simulink model "My_gfm_battery_sil_1_BS_2"  (R2018b)
settings: Solver=ode23t  StartTime=0.0  StopTime=30  MaxStep=1e-4  RelTol=1e-3
PreLoadFcn:
  | modelDir = fileparts(get_param(bdroot,'FileName'));
  | 
  | load_system(fullfile(modelDir,'controls_element_lib.slx'));
  | load_system(fullfile(modelDir,'test_sequence_lib.slx'));
InitFcn:
  | close all;
  | clear all;
  | clc;
  | 
  | % frequency nominals
  | F_NOM = 60;
  | W_NOM = 2 * pi * F_NOM;
  | 
  | % base values relative to inverter
  | % --------------------------------
  | VLL_INV_NOM = 480;
  | P_INV_NOM = 1e6;
  | Q_INV_NOM = 0.5e6;
  | S_INV_NOM = sqrt(P_INV_NOM^2 + Q_INV_NOM^2);
  | 
  | I_INV_BASE = S_INV_NOM/(sqrt(3)*VLL_INV_NOM);
  | Z_INV_BASE = VLL_INV_NOM^2/S_INV_NOM;
  | L_INV_BASE = Z_INV_BASE / W_NOM;
  | C_INV_BASE = 1 / (Z_INV_BASE * W_NOM);
  | 
  | % nominal ratings for power system model
  | % --------------------------------------
  | INVERTER_COUNT = 100;
  | 
  | VLV_NOM = VLL_INV_NOM;
  | VMV_NOM = 35e3;
  | VHV_NOM = 230e3;
  | S_PLANT = INVERTER_COUNT * S_INV_NOM;
  | 
  | N_GSU = VHV_NOM/VMV_NOM;
  | N_MVT = VMV_NOM/VLV_NOM;
  | 
  | I_LV_BASE = S_PLANT/(sqrt(3)*VLV_NOM);
  | I_MV_BASE = S_PLANT/(sqrt(3)*VMV_NOM);
  | I_HV_BASE = S_PLANT/(sqrt(3)*VHV_NOM);
  | 
  | Z_LV_BASE = VLV_NOM^2/S_PLANT;
  | Z_MV_BASE = VMV_NOM^2/S_PLANT;
  | Z_HV_BASE = VHV_NOM^2/S_PLANT;
  | 
  | L_LV_BASE = Z_LV_BASE / W_NOM;
  | L_MV_BASE = Z_MV_BASE / W_NOM;
  | L_HV_BASE = Z_HV_BASE / W_NOM;
  | C_LV_BASE = 1 / (Z_LV_BASE * W_NOM);
  | C_MV_BASE = 1 / (Z_MV_BASE * W_NOM);
  | C_HV_BASE = 1 / (Z_HV_BASE * W_NOM);
undefined symbols (not defined in the file): j, kpFastSync, kpSync, kpSyncFade, SRated, SyncFadeThres, tauBkSt, VllRated, wSync
libraries: simulink x59, test_sequence_lib x9, controls_element_lib x8
(part 4 of 7)

== system My_gfm_battery_sil_1_BS_2/My Inverter Controller /My_acChecks_A_V1/OV3 Timer ==
  note: Min one sample delay on Rise
  note: Max one sample delay on Fall
  in : Inport
  Constant : Constant  Value=T_STEP
  Constant1 : Constant  Value=0
  Constant2 : Constant  Value=TIMEOUT
  Constant3 : Constant  Value=T_STEP
  Gain : Gain  Gain=0
  Min1 : MinMax  Function=max  Inputs=2
  Min2 : MinMax  Inputs=2
  Relational Operator : RelationalOperator  Operator=>  OutDataTypeStr=boolean  RndMeth=Simplest
  Sum1 : Sum  Inputs=|++
  Sum2 : Sum  Inputs=|++
  Switch : Switch  Criteria=u2 > Threshold
  Unit Delay : UnitDelay  SampleTime=T_STEP
  out : Outport  VectorParamsAs1DForOutWhenUnconnected=on
  wires:
  Sum2/1 -> Relational Operator/1, Min2/1
  Sum1/1 -> Min2/2, Relational Operator/2
  Constant/1 -> Sum2/1
  Min2/1 -> Switch/1
  Constant1/1 -> Switch/3
  Unit Delay/1 -> Sum2/2
  in/1 -> Switch/2
  Switch/1 -> Unit Delay/1
  Relational Operator/1 -> out/1
  Min1/1 -> Sum1/1
  Constant2/1 -> Min1/1
  Constant3/1 -> Min1/2, Gain/1
  Gain/1 -> Sum1/2

== system My_gfm_battery_sil_1_BS_2/My Inverter Controller /My_acChecks_A_V1/UF1 Timer ==
  note: Min one sample delay on Rise
  note: Max one sample delay on Fall
  in : Inport
  Constant : Constant  Value=T_STEP
  Constant1 : Constant  Value=0
  Constant2 : Constant  Value=TIMEOUT
  Constant3 : Constant  Value=T_STEP
  Gain : Gain  Gain=0
  Min1 : MinMax  Function=max  Inputs=2
  Min2 : MinMax  Inputs=2
  Relational Operator : RelationalOperator  Operator=>  OutDataTypeStr=boolean  RndMeth=Simplest
  Sum1 : Sum  Inputs=|++
  Sum2 : Sum  Inputs=|++
  Switch : Switch  Criteria=u2 > Threshold
  Unit Delay : UnitDelay  SampleTime=T_STEP
  out : Outport  VectorParamsAs1DForOutWhenUnconnected=on
  wires:
  Sum2/1 -> Relational Operator/1, Min2/1
  Sum1/1 -> Min2/2, Relational Operator/2
  Constant/1 -> Sum2/1
  Min2/1 -> Switch/1
  Constant1/1 -> Switch/3
  Unit Delay/1 -> Sum2/2
  in/1 -> Switch/2
  Switch/1 -> Unit Delay/1
  Relational Operator/1 -> out/1
  Min1/1 -> Sum1/1
  Constant2/1 -> Min1/1
  Constant3/1 -> Min1/2, Gain/1
  Gain/1 -> Sum1/2

== system My_gfm_battery_sil_1_BS_2/My Inverter Controller /My_acChecks_A_V1/UF2 Timer ==
  note: Min one sample delay on Rise
  note: Max one sample delay on Fall
  in : Inport
  Constant : Constant  Value=T_STEP
  Constant1 : Constant  Value=0
  Constant2 : Constant  Value=TIMEOUT
  Constant3 : Constant  Value=T_STEP
  Gain : Gain  Gain=0
  Min1 : MinMax  Function=max  Inputs=2
  Min2 : MinMax  Inputs=2
  Relational Operator : RelationalOperator  Operator=>  OutDataTypeStr=boolean  RndMeth=Simplest
  Sum1 : Sum  Inputs=|++
  Sum2 : Sum  Inputs=|++
  Switch : Switch  Criteria=u2 > Threshold
  Unit Delay : UnitDelay  SampleTime=T_STEP
  out : Outport  VectorParamsAs1DForOutWhenUnconnected=on
  wires:
  Sum2/1 -> Relational Operator/1, Min2/1
  Sum1/1 -> Min2/2, Relational Operator/2
  Constant/1 -> Sum2/1
  Min2/1 -> Switch/1
  Constant1/1 -> Switch/3
  Unit Delay/1 -> Sum2/2
  in/1 -> Switch/2
  Switch/1 -> Unit Delay/1
  Relational Operator/1 -> out/1
  Min1/1 -> Sum1/1
  Constant2/1 -> Min1/1
  Constant3/1 -> Min1/2, Gain/1
  Gain/1 -> Sum1/2

== system My_gfm_battery_sil_1_BS_2/My Inverter Controller /My_acChecks_A_V1/UF3 Timer ==
  note: Min one sample delay on Rise
  note: Max one sample delay on Fall
  in : Inport
  Constant : Constant  Value=T_STEP
  Constant1 : Constant  Value=0
  Constant2 : Constant  Value=TIMEOUT
  Constant3 : Constant  Value=T_STEP
  Gain : Gain  Gain=0
  Min1 : MinMax  Function=max  Inputs=2
  Min2 : MinMax  Inputs=2
  Relational Operator : RelationalOperator  Operator=>  OutDataTypeStr=boolean  RndMeth=Simplest
  Sum1 : Sum  Inputs=|++
  Sum2 : Sum  Inputs=|++
  Switch : Switch  Criteria=u2 > Threshold
  Unit Delay : UnitDelay  SampleTime=T_STEP
  out : Outport  VectorParamsAs1DForOutWhenUnconnected=on
  wires:
  Sum2/1 -> Relational Operator/1, Min2/1
  Sum1/1 -> Min2/2, Relational Operator/2
  Constant/1 -> Sum2/1
  Min2/1 -> Switch/1
  Constant1/1 -> Switch/3
  Unit Delay/1 -> Sum2/2
  in/1 -> Switch/2
  Switch/1 -> Unit Delay/1
  Relational Operator/1 -> out/1
  Min1/1 -> Sum1/1
  Constant2/1 -> Min1/1
  Constant3/1 -> Min1/2, Gain/1
  Gain/1 -> Sum1/2

== system My_gfm_battery_sil_1_BS_2/My Inverter Controller /My_acChecks_A_V1/UV1 Timer ==
  note: Min one sample delay on Rise
  note: Max one sample delay on Fall
  in : Inport
  Constant : Constant  Value=T_STEP
  Constant1 : Constant  Value=0
  Constant2 : Constant  Value=TIMEOUT
  Constant3 : Constant  Value=T_STEP
  Gain : Gain  Gain=0
  Min1 : MinMax  Function=max  Inputs=2
  Min2 : MinMax  Inputs=2
  Relational Operator : RelationalOperator  Operator=>  OutDataTypeStr=boolean  RndMeth=Simplest
  Sum1 : Sum  Inputs=|++
  Sum2 : Sum  Inputs=|++
  Switch : Switch  Criteria=u2 > Threshold
  Unit Delay : UnitDelay  SampleTime=T_STEP
  out : Outport  VectorParamsAs1DForOutWhenUnconnected=on
  wires:
  Sum2/1 -> Relational Operator/1, Min2/1
  Sum1/1 -> Min2/2, Relational Operator/2
  Constant/1 -> Sum2/1
  Min2/1 -> Switch/1
  Constant1/1 -> Switch/3
  Unit Delay/1 -> Sum2/2
  in/1 -> Switch/2
  Switch/1 -> Unit Delay/1
  Relational Operator/1 -> out/1
  Min1/1 -> Sum1/1
  Constant2/1 -> Min1/1
  Constant3/1 -> Min1/2, Gain/1
  Gain/1 -> Sum1/2

== system My_gfm_battery_sil_1_BS_2/My Inverter Controller /My_acChecks_A_V1/UV2 Timer ==
  note: Min one sample delay on Rise
  note: Max one sample delay on Fall
  in : Inport
  Constant : Constant  Value=T_STEP
  Constant1 : Constant  Value=0
  Constant2 : Constant  Value=TIMEOUT
  Constant3 : Constant  Value=T_STEP
  Gain : Gain  Gain=0
  Min1 : MinMax  Function=max  Inputs=2
  Min2 : MinMax  Inputs=2
  Relational Operator : RelationalOperator  Operator=>  OutDataTypeStr=boolean  RndMeth=Simplest
  Sum1 : Sum  Inputs=|++
  Sum2 : Sum  Inputs=|++
  Switch : Switch  Criteria=u2 > Threshold
  Unit Delay : UnitDelay  SampleTime=T_STEP
  out : Outport  VectorParamsAs1DForOutWhenUnconnected=on
  wires:
  Sum2/1 -> Relational Operator/1, Min2/1
  Sum1/1 -> Min2/2, Relational Operator/2
  Constant/1 -> Sum2/1
  Min2/1 -> Switch/1
  Constant1/1 -> Switch/3
  Unit Delay/1 -> Sum2/2
  in/1 -> Switch/2
  Switch/1 -> Unit Delay/1
  Relational Operator/1 -> out/1
  Min1/1 -> Sum1/1
  Constant2/1 -> Min1/1
  Constant3/1 -> Min1/2, Gain/1
  Gain/1 -> Sum1/2

== system My_gfm_battery_sil_1_BS_2/My Inverter Controller /My_acChecks_A_V1/UV3 Timer ==
  note: Min one sample delay on Rise
  note: Max one sample delay on Fall
  in : Inport
  Constant : Constant  Value=T_STEP
  Constant1 : Constant  Value=0
  Constant2 : Constant  Value=TIMEOUT
  Constant3 : Constant  Value=T_STEP
  Gain : Gain  Gain=0
  Min1 : MinMax  Function=max  Inputs=2
  Min2 : MinMax  Inputs=2
  Relational Operator : RelationalOperator  Operator=>  OutDataTypeStr=boolean  RndMeth=Simplest
  Sum1 : Sum  Inputs=|++
  Sum2 : Sum  Inputs=|++
  Switch : Switch  Criteria=u2 > Threshold
  Unit Delay : UnitDelay  SampleTime=T_STEP
  out : Outport  VectorParamsAs1DForOutWhenUnconnected=on
  wires:
  Sum2/1 -> Relational Operator/1, Min2/1
  Sum1/1 -> Min2/2, Relational Operator/2
  Constant/1 -> Sum2/1
  Min2/1 -> Switch/1
  Constant1/1 -> Switch/3
  Unit Delay/1 -> Sum2/2
  in/1 -> Switch/2
  Switch/1 -> Unit Delay/1
  Relational Operator/1 -> out/1
  Min1/1 -> Sum1/1
  Constant2/1 -> Min1/1
  Constant3/1 -> Min1/2, Gain/1
  Gain/1 -> Sum1/2

== system My_gfm_battery_sil_1_BS_2/My Inverter Controller /My_acChecks_A_V2/Assert Timer ==
  note: Min one sample delay on Rise
  note: Max one sample delay on Fall
  in : Inport
  Constant : Constant  Value=T_STEP
  Constant1 : Constant  Value=0
  Constant2 : Constant  Value=TIMEOUT
  Constant3 : Constant  Value=T_STEP
  Gain : Gain  Gain=0
  Min1 : MinMax  Function=max  Inputs=2
  Min2 : MinMax  Inputs=2
  Relational Operator : RelationalOperator  Operator=>  OutDataTypeStr=boolean  RndMeth=Simplest
  Sum1 : Sum  Inputs=|++
  Sum2 : Sum  Inputs=|++
  Switch : Switch  Criteria=u2 > Threshold
  Unit Delay : UnitDelay  SampleTime=T_STEP
  out : Outport  VectorParamsAs1DForOutWhenUnconnected=on
  wires:
  Sum2/1 -> Relational Operator/1, Min2/1
  Sum1/1 -> Min2/2, Relational Operator/2
  Constant/1 -> Sum2/1
  Min2/1 -> Switch/1
  Constant1/1 -> Switch/3
  Unit Delay/1 -> Sum2/2
  in/1 -> Switch/2
  Switch/1 -> Unit Delay/1
  Relational Operator/1 -> out/1
  Min1/1 -> Sum1/1
  Constant2/1 -> Min1/1
  Constant3/1 -> Min1/2, Gain/1
  Gain/1 -> Sum1/2

== system My_gfm_battery_sil_1_BS_2/My Inverter Controller /My_acChecks_A_V2/Clear Timer1 ==
  note: Max one sample delay on Rise
  note: Min one sample delay on Fall
  in : Inport
  Constant : Constant  Value=T_STEP
  Constant1 : Constant  Value=0
  Constant2 : Constant  Value=TIMEOUT
  Constant3 : Constant  Value=T_STEP
  Min1 : MinMax  Function=max  Inputs=2
  Min2 : MinMax  Function=max  Inputs=2
  Relational Operator : RelationalOperator  Operator=>  OutDataTypeStr=boolean  RndMeth=Simplest
  Sum1 : Sum  Inputs=|++
  Sum2 : Sum  Inputs=|-+
  Switch : Switch  Criteria=u2 > Threshold
  Unit Delay : UnitDelay  InitialCondition=TIMER_INIT  SampleTime=T_STEP
  out : Outport  VectorParamsAs1DForOutWhenUnconnected=on
  wires:
  Sum1/1 -> Switch/1
  Sum2/1 -> Relational Operator/1, Min2/1
  Constant/1 -> Sum2/1
  Min2/1 -> Switch/3
  Constant1/1 -> Min2/2, Relational Operator/2
  Unit Delay/1 -> Sum2/2
  in/1 -> Switch/2
  Switch/1 -> Unit Delay/1
  Relational Operator/1 -> out/1
  Constant2/1 -> Min1/1
  Constant3/1 -> Min1/2, Sum1/2
  Min1/1 -> Sum1/1

== system My_gfm_battery_sil_1_BS_2/My Inverter Controller /My_acChecks_A_V2/Clear Timer10 ==
  note: Max one sample delay on Rise
  note: Min one sample delay on Fall
  in : Inport
  Constant : Constant  Value=T_STEP
  Constant1 : Constant  Value=0
  Constant2 : Constant  Value=TIMEOUT
  Constant3 : Constant  Value=T_STEP
  Min1 : MinMax  Function=max  Inputs=2
  Min2 : MinMax  Function=max  Inputs=2
  Relational Operator : RelationalOperator  Operator=>  OutDataTypeStr=boolean  RndMeth=Simplest
  Sum1 : Sum  Inputs=|++
  Sum2 : Sum  Inputs=|-+
  Switch : Switch  Criteria=u2 > Threshold
  Unit Delay : UnitDelay  InitialCondition=TIMER_INIT  SampleTime=T_STEP
  out : Outport  VectorParamsAs1DForOutWhenUnconnected=on
  wires:
  Sum1/1 -> Switch/1
  Sum2/1 -> Relational Operator/1, Min2/1
  Constant/1 -> Sum2/1
  Min2/1 -> Switch/3
  Constant1/1 -> Min2/2, Relational Operator/2
  Unit Delay/1 -> Sum2/2
  in/1 -> Switch/2
  Switch/1 -> Unit Delay/1
  Relational Operator/1 -> out/1
  Constant2/1 -> Min1/1
  Constant3/1 -> Min1/2, Sum1/2
  Min1/1 -> Sum1/1

== system My_gfm_battery_sil_1_BS_2/My Inverter Controller /My_acChecks_A_V2/Clear Timer11 ==
  note: Max one sample delay on Rise
  note: Min one sample delay on Fall
  in : Inport
  Constant : Constant  Value=T_STEP
  Constant1 : Constant  Value=0
  Constant2 : Constant  Value=TIMEOUT
  Constant3 : Constant  Value=T_STEP
  Min1 : MinMax  Function=max  Inputs=2
  Min2 : MinMax  Function=max  Inputs=2
  Relational Operator : RelationalOperator  Operator=>  OutDataTypeStr=boolean  RndMeth=Simplest
  Sum1 : Sum  Inputs=|++
  Sum2 : Sum  Inputs=|-+
  Switch : Switch  Criteria=u2 > Threshold
  Unit Delay : UnitDelay  InitialCondition=TIMER_INIT  SampleTime=T_STEP
  out : Outport  VectorParamsAs1DForOutWhenUnconnected=on
  wires:
  Sum1/1 -> Switch/1
  Sum2/1 -> Relational Operator/1, Min2/1
  Constant/1 -> Sum2/1
  Min2/1 -> Switch/3
  Constant1/1 -> Min2/2, Relational Operator/2
  Unit Delay/1 -> Sum2/2
  in/1 -> Switch/2
  Switch/1 -> Unit Delay/1
  Relational Operator/1 -> out/1
  Constant2/1 -> Min1/1
  Constant3/1 -> Min1/2, Sum1/2
  Min1/1 -> Sum1/1

== system My_gfm_battery_sil_1_BS_2/My Inverter Controller /My_acChecks_A_V2/Clear Timer12 ==
  note: Max one sample delay on Rise
  note: Min one sample delay on Fall
  in : Inport
  Constant : Constant  Value=T_STEP
  Constant1 : Constant  Value=0
  Constant2 : Constant  Value=TIMEOUT
  Constant3 : Constant  Value=T_STEP
  Min1 : MinMax  Function=max  Inputs=2
  Min2 : MinMax  Function=max  Inputs=2
  Relational Operator : RelationalOperator  Operator=>  OutDataTypeStr=boolean  RndMeth=Simplest
  Sum1 : Sum  Inputs=|++
  Sum2 : Sum  Inputs=|-+
  Switch : Switch  Criteria=u2 > Threshold
  Unit Delay : UnitDelay  InitialCondition=TIMER_INIT  SampleTime=T_STEP
  out : Outport  VectorParamsAs1DForOutWhenUnconnected=on
  wires:
  Sum1/1 -> Switch/1
  Sum2/1 -> Relational Operator/1, Min2/1
  Constant/1 -> Sum2/1
  Min2/1 -> Switch/3
  Constant1/1 -> Min2/2, Relational Operator/2
  Unit Delay/1 -> Sum2/2
  in/1 -> Switch/2
  Switch/1 -> Unit Delay/1
  Relational Operator/1 -> out/1
  Constant2/1 -> Min1/1
  Constant3/1 -> Min1/2, Sum1/2
  Min1/1 -> Sum1/1

== system My_gfm_battery_sil_1_BS_2/My Inverter Controller /My_acChecks_A_V2/Clear Timer13 ==
  note: Max one sample delay on Rise
  note: Min one sample delay on Fall
  in : Inport
  Constant : Constant  Value=T_STEP
  Constant1 : Constant  Value=0
  Constant2 : Constant  Value=TIMEOUT
  Constant3 : Constant  Value=T_STEP
  Min1 : MinMax  Function=max  Inputs=2
  Min2 : MinMax  Function=max  Inputs=2
  Relational Operator : RelationalOperator  Operator=>  OutDataTypeStr=boolean  RndMeth=Simplest
  Sum1 : Sum  Inputs=|++
  Sum2 : Sum  Inputs=|-+
  Switch : Switch  Criteria=u2 > Threshold
  Unit Delay : UnitDelay  InitialCondition=TIMER_INIT  SampleTime=T_STEP
  out : Outport  VectorParamsAs1DForOutWhenUnconnected=on
  wires:
  Sum1/1 -> Switch/1
  Sum2/1 -> Relational Operator/1, Min2/1
  Constant/1 -> Sum2/1
  Min2/1 -> Switch/3
  Constant1/1 -> Min2/2, Relational Operator/2
  Unit Delay/1 -> Sum2/2
  in/1 -> Switch/2
  Switch/1 -> Unit Delay/1
  Relational Operator/1 -> out/1
  Constant2/1 -> Min1/1
  Constant3/1 -> Min1/2, Sum1/2
  Min1/1 -> Sum1/1

== system My_gfm_battery_sil_1_BS_2/My Inverter Controller /My_acChecks_A_V2/Clear Timer14 ==
  note: Max one sample delay on Rise
  note: Min one sample delay on Fall
  in : Inport
  Constant : Constant  Value=T_STEP
  Constant1 : Constant  Value=0
  Constant2 : Constant  Value=TIMEOUT
  Constant3 : Constant  Value=T_STEP
  Min1 : MinMax  Function=max  Inputs=2
  Min2 : MinMax  Function=max  Inputs=2
  Relational Operator : RelationalOperator  Operator=>  OutDataTypeStr=boolean  RndMeth=Simplest
  Sum1 : Sum  Inputs=|++
  Sum2 : Sum  Inputs=|-+
  Switch : Switch  Criteria=u2 > Threshold
  Unit Delay : UnitDelay  InitialCondition=TIMER_INIT  SampleTime=T_STEP
  out : Outport  VectorParamsAs1DForOutWhenUnconnected=on
  wires:
  Sum1/1 -> Switch/1
  Sum2/1 -> Relational Operator/1, Min2/1
  Constant/1 -> Sum2/1
  Min2/1 -> Switch/3
  Constant1/1 -> Min2/2, Relational Operator/2
  Unit Delay/1 -> Sum2/2
  in/1 -> Switch/2
  Switch/1 -> Unit Delay/1
  Relational Operator/1 -> out/1
  Constant2/1 -> Min1/1
  Constant3/1 -> Min1/2, Sum1/2
  Min1/1 -> Sum1/1

== system My_gfm_battery_sil_1_BS_2/My Inverter Controller /My_acChecks_A_V2/Clear Timer15 ==
  note: Max one sample delay on Rise
  note: Min one sample delay on Fall
  in : Inport
  Constant : Constant  Value=T_STEP
  Constant1 : Constant  Value=0
  Constant2 : Constant  Value=TIMEOUT
  Constant3 : Constant  Value=T_STEP
  Min1 : MinMax  Function=max  Inputs=2
  Min2 : MinMax  Function=max  Inputs=2
  Relational Operator : RelationalOperator  Operator=>  OutDataTypeStr=boolean  RndMeth=Simplest
  Sum1 : Sum  Inputs=|++
  Sum2 : Sum  Inputs=|-+
  Switch : Switch  Criteria=u2 > Threshold
  Unit Delay : UnitDelay  InitialCondition=TIMER_INIT  SampleTime=T_STEP
  out : Outport  VectorParamsAs1DForOutWhenUnconnected=on
  wires:
  Sum1/1 -> Switch/1
  Sum2/1 -> Relational Operator/1, Min2/1
  Constant/1 -> Sum2/1
  Min2/1 -> Switch/3
  Constant1/1 -> Min2/2, Relational Operator/2
  Unit Delay/1 -> Sum2/2
  in/1 -> Switch/2
  Switch/1 -> Unit Delay/1
  Relational Operator/1 -> out/1
  Constant2/1 -> Min1/1
  Constant3/1 -> Min1/2, Sum1/2
  Min1/1 -> Sum1/1

== system My_gfm_battery_sil_1_BS_2/My Inverter Controller /My_acChecks_A_V2/Clear Timer2 ==
  note: Max one sample delay on Rise
  note: Min one sample delay on Fall
  in : Inport
  Constant : Constant  Value=T_STEP
  Constant1 : Constant  Value=0
  Constant2 : Constant  Value=TIMEOUT
  Constant3 : Constant  Value=T_STEP
  Min1 : MinMax  Function=max  Inputs=2
  Min2 : MinMax  Function=max  Inputs=2
  Relational Operator : RelationalOperator  Operator=>  OutDataTypeStr=boolean  RndMeth=Simplest
  Sum1 : Sum  Inputs=|++
  Sum2 : Sum  Inputs=|-+
  Switch : Switch  Criteria=u2 > Threshold
  Unit Delay : UnitDelay  InitialCondition=TIMER_INIT  SampleTime=T_STEP
  out : Outport  VectorParamsAs1DForOutWhenUnconnected=on
  wires:
  Sum1/1 -> Switch/1
  Sum2/1 -> Relational Operator/1, Min2/1
  Constant/1 -> Sum2/1
  Min2/1 -> Switch/3
  Constant1/1 -> Min2/2, Relational Operator/2
  Unit Delay/1 -> Sum2/2
  in/1 -> Switch/2
  Switch/1 -> Unit Delay/1
  Relational Operator/1 -> out/1
  Constant2/1 -> Min1/1
  Constant3/1 -> Min1/2, Sum1/2
  Min1/1 -> Sum1/1

== system My_gfm_battery_sil_1_BS_2/My Inverter Controller /My_acChecks_A_V2/Clear Timer3 ==
  note: Max one sample delay on Rise
  note: Min one sample delay on Fall
  in : Inport
  Constant : Constant  Value=T_STEP
  Constant1 : Constant  Value=0
  Constant2 : Constant  Value=TIMEOUT
  Constant3 : Constant  Value=T_STEP
  Min1 : MinMax  Function=max  Inputs=2
  Min2 : MinMax  Function=max  Inputs=2
  Relational Operator : RelationalOperator  Operator=>  OutDataTypeStr=boolean  RndMeth=Simplest
  Sum1 : Sum  Inputs=|++
  Sum2 : Sum  Inputs=|-+
  Switch : Switch  Criteria=u2 > Threshold
  Unit Delay : UnitDelay  InitialCondition=TIMER_INIT  SampleTime=T_STEP
  out : Outport  VectorParamsAs1DForOutWhenUnconnected=on
  wires:
  Sum1/1 -> Switch/1
  Sum2/1 -> Relational Operator/1, Min2/1
  Constant/1 -> Sum2/1
  Min2/1 -> Switch/3
  Constant1/1 -> Min2/2, Relational Operator/2
  Unit Delay/1 -> Sum2/2
  in/1 -> Switch/2
  Switch/1 -> Unit Delay/1
  Relational Operator/1 -> out/1
  Constant2/1 -> Min1/1
  Constant3/1 -> Min1/2, Sum1/2
  Min1/1 -> Sum1/1

== system My_gfm_battery_sil_1_BS_2/My Inverter Controller /My_acChecks_A_V2/Clear Timer4 ==
  note: Max one sample delay on Rise
  note: Min one sample delay on Fall
  in : Inport
  Constant : Constant  Value=T_STEP
  Constant1 : Constant  Value=0
  Constant2 : Constant  Value=TIMEOUT
  Constant3 : Constant  Value=T_STEP
  Min1 : MinMax  Function=max  Inputs=2
  Min2 : MinMax  Function=max  Inputs=2
  Relational Operator : RelationalOperator  Operator=>  OutDataTypeStr=boolean  RndMeth=Simplest
  Sum1 : Sum  Inputs=|++
  Sum2 : Sum  Inputs=|-+
  Switch : Switch  Criteria=u2 > Threshold
  Unit Delay : UnitDelay  InitialCondition=TIMER_INIT  SampleTime=T_STEP
  out : Outport  VectorParamsAs1DForOutWhenUnconnected=on
  wires:
  Sum1/1 -> Switch/1
  Sum2/1 -> Relational Operator/1, Min2/1
  Constant/1 -> Sum2/1
  Min2/1 -> Switch/3
  Constant1/1 -> Min2/2, Relational Operator/2
  Unit Delay/1 -> Sum2/2
  in/1 -> Switch/2
  Switch/1 -> Unit Delay/1
  Relational Operator/1 -> out/1
  Constant2/1 -> Min1/1
  Constant3/1 -> Min1/2, Sum1/2
  Min1/1 -> Sum1/1

== system My_gfm_battery_sil_1_BS_2/My Inverter Controller /My_acChecks_A_V2/Clear Timer5 ==
  note: Max one sample delay on Rise
  note: Min one sample delay on Fall
  in : Inport
  Constant : Constant  Value=T_STEP
  Constant1 : Constant  Value=0
  Constant2 : Constant  Value=TIMEOUT
  Constant3 : Constant  Value=T_STEP
  Min1 : MinMax  Function=max  Inputs=2
  Min2 : MinMax  Function=max  Inputs=2
  Relational Operator : RelationalOperator  Operator=>  OutDataTypeStr=boolean  RndMeth=Simplest
  Sum1 : Sum  Inputs=|++
  Sum2 : Sum  Inputs=|-+
  Switch : Switch  Criteria=u2 > Threshold
  Unit Delay : UnitDelay  InitialCondition=TIMER_INIT  SampleTime=T_STEP
  out : Outport  VectorParamsAs1DForOutWhenUnconnected=on
  wires:
  Sum1/1 -> Switch/1
  Sum2/1 -> Relational Operator/1, Min2/1
  Constant/1 -> Sum2/1
  Min2/1 -> Switch/3
  Constant1/1 -> Min2/2, Relational Operator/2
  Unit Delay/1 -> Sum2/2
  in/1 -> Switch/2
  Switch/1 -> Unit Delay/1
  Relational Operator/1 -> out/1
  Constant2/1 -> Min1/1
  Constant3/1 -> Min1/2, Sum1/2
  Min1/1 -> Sum1/1

== system My_gfm_battery_sil_1_BS_2/My Inverter Controller /My_acChecks_A_V2/Clear Timer6 ==
  note: Max one sample delay on Rise
  note: Min one sample delay on Fall
  in : Inport
  Constant : Constant  Value=T_STEP
  Constant1 : Constant  Value=0
  Constant2 : Constant  Value=TIMEOUT
  Constant3 : Constant  Value=T_STEP
  Min1 : MinMax  Function=max  Inputs=2
  Min2 : MinMax  Function=max  Inputs=2
  Relational Operator : RelationalOperator  Operator=>  OutDataTypeStr=boolean  RndMeth=Simplest
  Sum1 : Sum  Inputs=|++
  Sum2 : Sum  Inputs=|-+
  Switch : Switch  Criteria=u2 > Threshold
  Unit Delay : UnitDelay  InitialCondition=TIMER_INIT  SampleTime=T_STEP
  out : Outport  VectorParamsAs1DForOutWhenUnconnected=on
  wires:
  Sum1/1 -> Switch/1
  Sum2/1 -> Relational Operator/1, Min2/1
  Constant/1 -> Sum2/1
  Min2/1 -> Switch/3
  Constant1/1 -> Min2/2, Relational Operator/2
  Unit Delay/1 -> Sum2/2
  in/1 -> Switch/2
  Switch/1 -> Unit Delay/1
  Relational Operator/1 -> out/1
  Constant2/1 -> Min1/1
  Constant3/1 -> Min1/2, Sum1/2
  Min1/1 -> Sum1/1

== system My_gfm_battery_sil_1_BS_2/My Inverter Controller /My_acChecks_A_V2/Clear Timer7 ==
  note: Max one sample delay on Rise
  note: Min one sample delay on Fall
  in : Inport
  Constant : Constant  Value=T_STEP
  Constant1 : Constant  Value=0
  Constant2 : Constant  Value=TIMEOUT
  Constant3 : Constant  Value=T_STEP
  Min1 : MinMax  Function=max  Inputs=2
  Min2 : MinMax  Function=max  Inputs=2
  Relational Operator : RelationalOperator  Operator=>  OutDataTypeStr=boolean  RndMeth=Simplest
  Sum1 : Sum  Inputs=|++
  Sum2 : Sum  Inputs=|-+
  Switch : Switch  Criteria=u2 > Threshold
  Unit Delay : UnitDelay  InitialCondition=TIMER_INIT  SampleTime=T_STEP
  out : Outport  VectorParamsAs1DForOutWhenUnconnected=on
  wires:
  Sum1/1 -> Switch/1
  Sum2/1 -> Relational Operator/1, Min2/1
  Constant/1 -> Sum2/1
  Min2/1 -> Switch/3
  Constant1/1 -> Min2/2, Relational Operator/2
  Unit Delay/1 -> Sum2/2
  in/1 -> Switch/2
  Switch/1 -> Unit Delay/1
  Relational Operator/1 -> out/1
  Constant2/1 -> Min1/1
  Constant3/1 -> Min1/2, Sum1/2
  Min1/1 -> Sum1/1

== system My_gfm_battery_sil_1_BS_2/My Inverter Controller /My_acChecks_A_V2/Clear Timer8 ==
  note: Max one sample delay on Rise
  note: Min one sample delay on Fall
  in : Inport
  Constant : Constant  Value=T_STEP
  Constant1 : Constant  Value=0
  Constant2 : Constant  Value=TIMEOUT
  Constant3 : Constant  Value=T_STEP
  Min1 : MinMax  Function=max  Inputs=2
  Min2 : MinMax  Function=max  Inputs=2
  Relational Operator : RelationalOperator  Operator=>  OutDataTypeStr=boolean  RndMeth=Simplest
  Sum1 : Sum  Inputs=|++
  Sum2 : Sum  Inputs=|-+
  Switch : Switch  Criteria=u2 > Threshold
  Unit Delay : UnitDelay  InitialCondition=TIMER_INIT  SampleTime=T_STEP
  out : Outport  VectorParamsAs1DForOutWhenUnconnected=on
  wires:
  Sum1/1 -> Switch/1
  Sum2/1 -> Relational Operator/1, Min2/1
  Constant/1 -> Sum2/1
  Min2/1 -> Switch/3
  Constant1/1 -> Min2/2, Relational Operator/2
  Unit Delay/1 -> Sum2/2
  in/1 -> Switch/2
  Switch/1 -> Unit Delay/1
  Relational Operator/1 -> out/1
  Constant2/1 -> Min1/1
  Constant3/1 -> Min1/2, Sum1/2
  Min1/1 -> Sum1/1

== system My_gfm_battery_sil_1_BS_2/My Inverter Controller /My_acChecks_A_V2/Clear Timer9 ==
  note: Max one sample delay on Rise
  note: Min one sample delay on Fall
  in : Inport
  Constant : Constant  Value=T_STEP
  Constant1 : Constant  Value=0
  Constant2 : Constant  Value=TIMEOUT
  Constant3 : Constant  Value=T_STEP
  Min1 : MinMax  Function=max  Inputs=2
  Min2 : MinMax  Function=max  Inputs=2
  Relational Operator : RelationalOperator  Operator=>  OutDataTypeStr=boolean  RndMeth=Simplest
  Sum1 : Sum  Inputs=|++
  Sum2 : Sum  Inputs=|-+
  Switch : Switch  Criteria=u2 > Threshold
  Unit Delay : UnitDelay  InitialCondition=TIMER_INIT  SampleTime=T_STEP
  out : Outport  VectorParamsAs1DForOutWhenUnconnected=on
  wires:
  Sum1/1 -> Switch/1
  Sum2/1 -> Relational Operator/1, Min2/1
  Constant/1 -> Sum2/1
  Min2/1 -> Switch/3
  Constant1/1 -> Min2/2, Relational Operator/2
  Unit Delay/1 -> Sum2/2
  in/1 -> Switch/2
  Switch/1 -> Unit Delay/1
  Relational Operator/1 -> out/1
  Constant2/1 -> Min1/1
  Constant3/1 -> Min1/2, Sum1/2
  Min1/1 -> Sum1/1

== system My_gfm_battery_sil_1_BS_2/My Inverter Controller /My_acChecks_A_V2/OF1 Timer ==
  note: Min one sample delay on Rise
  note: Max one sample delay on Fall
  in : Inport
  Constant : Constant  Value=T_STEP
  Constant1 : Constant  Value=0
  Constant2 : Constant  Value=TIMEOUT
  Constant3 : Constant  Value=T_STEP
  Gain : Gain  Gain=0
  Min1 : MinMax  Function=max  Inputs=2
  Min2 : MinMax  Inputs=2
  Relational Operator : RelationalOperator  Operator=>  OutDataTypeStr=boolean  RndMeth=Simplest
  Sum1 : Sum  Inputs=|++
  Sum2 : Sum  Inputs=|++
  Switch : Switch  Criteria=u2 > Threshold
  Unit Delay : UnitDelay  SampleTime=T_STEP
  out : Outport  VectorParamsAs1DForOutWhenUnconnected=on
  wires:
  Sum2/1 -> Relational Operator/1, Min2/1
  Sum1/1 -> Min2/2, Relational Operator/2
  Constant/1 -> Sum2/1
  Min2/1 -> Switch/1
  Constant1/1 -> Switch/3
  Unit Delay/1 -> Sum2/2
  in/1 -> Switch/2
  Switch/1 -> Unit Delay/1
  Relational Operator/1 -> out/1
  Min1/1 -> Sum1/1
  Constant2/1 -> Min1/1
  Constant3/1 -> Min1/2, Gain/1
  Gain/1 -> Sum1/2

== system My_gfm_battery_sil_1_BS_2/My Inverter Controller /My_acChecks_A_V2/OF2 Timer ==
  note: Min one sample delay on Rise
  note: Max one sample delay on Fall
  in : Inport
  Constant : Constant  Value=T_STEP
  Constant1 : Constant  Value=0
  Constant2 : Constant  Value=TIMEOUT
  Constant3 : Constant  Value=T_STEP
  Gain : Gain  Gain=0
  Min1 : MinMax  Function=max  Inputs=2
  Min2 : MinMax  Inputs=2
  Relational Operator : RelationalOperator  Operator=>  OutDataTypeStr=boolean  RndMeth=Simplest
  Sum1 : Sum  Inputs=|++
  Sum2 : Sum  Inputs=|++
  Switch : Switch  Criteria=u2 > Threshold
  Unit Delay : UnitDelay  SampleTime=T_STEP
  out : Outport  VectorParamsAs1DForOutWhenUnconnected=on
  wires:
  Sum2/1 -> Relational Operator/1, Min2/1
  Sum1/1 -> Min2/2, Relational Operator/2
  Constant/1 -> Sum2/1
  Min2/1 -> Switch/1
  Constant1/1 -> Switch/3
  Unit Delay/1 -> Sum2/2
  in/1 -> Switch/2
  Switch/1 -> Unit Delay/1
  Relational Operator/1 -> out/1
  Min1/1 -> Sum1/1
  Constant2/1 -> Min1/1
  Constant3/1 -> Min1/2, Gain/1
  Gain/1 -> Sum1/2

== system My_gfm_battery_sil_1_BS_2/My Inverter Controller /My_acChecks_A_V2/OF3 Timer ==
  note: Min one sample delay on Rise
  note: Max one sample delay on Fall
  in : Inport
  Constant : Constant  Value=T_STEP
  Constant1 : Constant  Value=0
  Constant2 : Constant  Value=TIMEOUT
  Constant3 : Constant  Value=T_STEP
  Gain : Gain  Gain=0
  Min1 : MinMax  Function=max  Inputs=2
  Min2 : MinMax  Inputs=2
  Relational Operator : RelationalOperator  Operator=>  OutDataTypeStr=boolean  RndMeth=Simplest
  Sum1 : Sum  Inputs=|++
  Sum2 : Sum  Inputs=|++
  Switch : Switch  Criteria=u2 > Threshold
  Unit Delay : UnitDelay  SampleTime=T_STEP
  out : Outport  VectorParamsAs1DForOutWhenUnconnected=on
  wires:
  Sum2/1 -> Relational Operator/1, Min2/1
  Sum1/1 -> Min2/2, Relational Operator/2
  Constant/1 -> Sum2/1
  Min2/1 -> Switch/1
  Constant1/1 -> Switch/3
  Unit Delay/1 -> Sum2/2
  in/1 -> Switch/2
  Switch/1 -> Unit Delay/1
  Relational Operator/1 -> out/1
  Min1/1 -> Sum1/1
  Constant2/1 -> Min1/1
  Constant3/1 -> Min1/2, Gain/1
  Gain/1 -> Sum1/2

== system My_gfm_battery_sil_1_BS_2/My Inverter Controller /My_acChecks_A_V2/OV1 Timer ==
  note: Min one sample delay on Rise
  note: Max one sample delay on Fall
  in : Inport
  Constant : Constant  Value=T_STEP
  Constant1 : Constant  Value=0
  Constant2 : Constant  Value=TIMEOUT
  Constant3 : Constant  Value=T_STEP
  Gain : Gain  Gain=0
  Min1 : MinMax  Function=max  Inputs=2
  Min2 : MinMax  Inputs=2
  Relational Operator : RelationalOperator  Operator=>  OutDataTypeStr=boolean  RndMeth=Simplest
  Sum1 : Sum  Inputs=|++
  Sum2 : Sum  Inputs=|++
  Switch : Switch  Criteria=u2 > Threshold
  Unit Delay : UnitDelay  SampleTime=T_STEP
  out : Outport  VectorParamsAs1DForOutWhenUnconnected=on
  wires:
  Sum2/1 -> Relational Operator/1, Min2/1
  Sum1/1 -> Min2/2, Relational Operator/2
  Constant/1 -> Sum2/1
  Min2/1 -> Switch/1
  Constant1/1 -> Switch/3
  Unit Delay/1 -> Sum2/2
  in/1 -> Switch/2
  Switch/1 -> Unit Delay/1
  Relational Operator/1 -> out/1
  Min1/1 -> Sum1/1
  Constant2/1 -> Min1/1
  Constant3/1 -> Min1/2, Gain/1
  Gain/1 -> Sum1/2

== system My_gfm_battery_sil_1_BS_2/My Inverter Controller /My_acChecks_A_V2/OV2 Timer ==
  note: Min one sample delay on Rise
  note: Max one sample delay on Fall
  in : Inport
  Constant : Constant  Value=T_STEP
  Constant1 : Constant  Value=0
  Constant2 : Constant  Value=TIMEOUT
  Constant3 : Constant  Value=T_STEP
  Gain : Gain  Gain=0
  Min1 : MinMax  Function=max  Inputs=2
  Min2 : MinMax  Inputs=2
  Relational Operator : RelationalOperator  Operator=>  OutDataTypeStr=boolean  RndMeth=Simplest
  Sum1 : Sum  Inputs=|++
  Sum2 : Sum  Inputs=|++
  Switch : Switch  Criteria=u2 > Threshold
  Unit Delay : UnitDelay  SampleTime=T_STEP
  out : Outport  VectorParamsAs1DForOutWhenUnconnected=on
  wires:
  Sum2/1 -> Relational Operator/1, Min2/1
  Sum1/1 -> Min2/2, Relational Operator/2
  Constant/1 -> Sum2/1
  Min2/1 -> Switch/1
  Constant1/1 -> Switch/3
  Unit Delay/1 -> Sum2/2
  in/1 -> Switch/2
  Switch/1 -> Unit Delay/1
  Relational Operator/1 -> out/1
  Min1/1 -> Sum1/1
  Constant2/1 -> Min1/1
  Constant3/1 -> Min1/2, Gain/1
  Gain/1 -> Sum1/2

== system My_gfm_battery_sil_1_BS_2/My Inverter Controller /My_acChecks_A_V2/OV3 Timer ==
  note: Min one sample delay on Rise
  note: Max one sample delay on Fall
  in : Inport
  Constant : Constant  Value=T_STEP
  Constant1 : Constant  Value=0
  Constant2 : Constant  Value=TIMEOUT
  Constant3 : Constant  Value=T_STEP
  Gain : Gain  Gain=0
  Min1 : MinMax  Function=max  Inputs=2
  Min2 : MinMax  Inputs=2
  Relational Operator : RelationalOperator  Operator=>  OutDataTypeStr=boolean  RndMeth=Simplest
  Sum1 : Sum  Inputs=|++
  Sum2 : Sum  Inputs=|++
  Switch : Switch  Criteria=u2 > Threshold
  Unit Delay : UnitDelay  SampleTime=T_STEP
  out : Outport  VectorParamsAs1DForOutWhenUnconnected=on
  wires:
  Sum2/1 -> Relational Operator/1, Min2/1
  Sum1/1 -> Min2/2, Relational Operator/2
  Constant/1 -> Sum2/1
  Min2/1 -> Switch/1
  Constant1/1 -> Switch/3
  Unit Delay/1 -> Sum2/2
  in/1 -> Switch/2
  Switch/1 -> Unit Delay/1
  Relational Operator/1 -> out/1
  Min1/1 -> Sum1/1
  Constant2/1 -> Min1/1
  Constant3/1 -> Min1/2, Gain/1
  Gain/1 -> Sum1/2

== system My_gfm_battery_sil_1_BS_2/My Inverter Controller /My_acChecks_A_V2/UF1 Timer ==
  note: Min one sample delay on Rise
  note: Max one sample delay on Fall
  in : Inport
  Constant : Constant  Value=T_STEP
  Constant1 : Constant  Value=0
  Constant2 : Constant  Value=TIMEOUT
  Constant3 : Constant  Value=T_STEP
  Gain : Gain  Gain=0
  Min1 : MinMax  Function=max  Inputs=2
  Min2 : MinMax  Inputs=2
  Relational Operator : RelationalOperator  Operator=>  OutDataTypeStr=boolean  RndMeth=Simplest
  Sum1 : Sum  Inputs=|++
  Sum2 : Sum  Inputs=|++
  Switch : Switch  Criteria=u2 > Threshold
  Unit Delay : UnitDelay  SampleTime=T_STEP
  out : Outport  VectorParamsAs1DForOutWhenUnconnected=on
  wires:
  Sum2/1 -> Relational Operator/1, Min2/1
  Sum1/1 -> Min2/2, Relational Operator/2
  Constant/1 -> Sum2/1
  Min2/1 -> Switch/1
  Constant1/1 -> Switch/3
  Unit Delay/1 -> Sum2/2
  in/1 -> Switch/2
  Switch/1 -> Unit Delay/1
  Relational Operator/1 -> out/1
  Min1/1 -> Sum1/1
  Constant2/1 -> Min1/1
  Constant3/1 -> Min1/2, Gain/1
  Gain/1 -> Sum1/2

== system My_gfm_battery_sil_1_BS_2/My Inverter Controller /My_acChecks_A_V2/UF2 Timer ==
  note: Min one sample delay on Rise
  note: Max one sample delay on Fall
  in : Inport
  Constant : Constant  Value=T_STEP
  Constant1 : Constant  Value=0
  Constant2 : Constant  Value=TIMEOUT
  Constant3 : Constant  Value=T_STEP
  Gain : Gain  Gain=0
  Min1 : MinMax  Function=max  Inputs=2
  Min2 : MinMax  Inputs=2
  Relational Operator : RelationalOperator  Operator=>  OutDataTypeStr=boolean  RndMeth=Simplest
  Sum1 : Sum  Inputs=|++
  Sum2 : Sum  Inputs=|++
  Switch : Switch  Criteria=u2 > Threshold
  Unit Delay : UnitDelay  SampleTime=T_STEP
  out : Outport  VectorParamsAs1DForOutWhenUnconnected=on
  wires:
  Sum2/1 -> Relational Operator/1, Min2/1
  Sum1/1 -> Min2/2, Relational Operator/2
  Constant/1 -> Sum2/1
  Min2/1 -> Switch/1
  Constant1/1 -> Switch/3
  Unit Delay/1 -> Sum2/2
  in/1 -> Switch/2
  Switch/1 -> Unit Delay/1
  Relational Operator/1 -> out/1
  Min1/1 -> Sum1/1
  Constant2/1 -> Min1/1
  Constant3/1 -> Min1/2, Gain/1
  Gain/1 -> Sum1/2

== system My_gfm_battery_sil_1_BS_2/My Inverter Controller /My_acChecks_A_V2/UF3 Timer ==
  note: Min one sample delay on Rise
  note: Max one sample delay on Fall
  in : Inport
  Constant : Constant  Value=T_STEP
  Constant1 : Constant  Value=0
  Constant2 : Constant  Value=TIMEOUT
  Constant3 : Constant  Value=T_STEP
  Gain : Gain  Gain=0
  Min1 : MinMax  Function=max  Inputs=2
  Min2 : MinMax  Inputs=2
  Relational Operator : RelationalOperator  Operator=>  OutDataTypeStr=boolean  RndMeth=Simplest
  Sum1 : Sum  Inputs=|++
  Sum2 : Sum  Inputs=|++
  Switch : Switch  Criteria=u2 > Threshold
  Unit Delay : UnitDelay  SampleTime=T_STEP
  out : Outport  VectorParamsAs1DForOutWhenUnconnected=on
  wires:
  Sum2/1 -> Relational Operator/1, Min2/1
  Sum1/1 -> Min2/2, Relational Operator/2
  Constant/1 -> Sum2/1
  Min2/1 -> Switch/1
  Constant1/1 -> Switch/3
  Unit Delay/1 -> Sum2/2
  in/1 -> Switch/2
  Switch/1 -> Unit Delay/1
  Relational Operator/1 -> out/1
  Min1/1 -> Sum1/1
  Constant2/1 -> Min1/1
  Constant3/1 -> Min1/2, Gain/1
  Gain/1 -> Sum1/2

== system My_gfm_battery_sil_1_BS_2/My Inverter Controller /My_acChecks_A_V2/UV1 Timer ==
  note: Min one sample delay on Rise
  note: Max one sample delay on Fall
  in : Inport
  Constant : Constant  Value=T_STEP
  Constant1 : Constant  Value=0
  Constant2 : Constant  Value=TIMEOUT
  Constant3 : Constant  Value=T_STEP
  Gain : Gain  Gain=0
  Min1 : MinMax  Function=max  Inputs=2
  Min2 : MinMax  Inputs=2
  Relational Operator : RelationalOperator  Operator=>  OutDataTypeStr=boolean  RndMeth=Simplest
  Sum1 : Sum  Inputs=|++
  Sum2 : Sum  Inputs=|++
  Switch : Switch  Criteria=u2 > Threshold
  Unit Delay : UnitDelay  SampleTime=T_STEP
  out : Outport  VectorParamsAs1DForOutWhenUnconnected=on
  wires:
  Sum2/1 -> Relational Operator/1, Min2/1
  Sum1/1 -> Min2/2, Relational Operator/2
  Constant/1 -> Sum2/1
  Min2/1 -> Switch/1
  Constant1/1 -> Switch/3
  Unit Delay/1 -> Sum2/2
  in/1 -> Switch/2
  Switch/1 -> Unit Delay/1
  Relational Operator/1 -> out/1
  Min1/1 -> Sum1/1
  Constant2/1 -> Min1/1
  Constant3/1 -> Min1/2, Gain/1
  Gain/1 -> Sum1/2

== system My_gfm_battery_sil_1_BS_2/My Inverter Controller /My_acChecks_A_V2/UV2 Timer ==
  note: Min one sample delay on Rise
  note: Max one sample delay on Fall
  in : Inport
  Constant : Constant  Value=T_STEP
  Constant1 : Constant  Value=0
  Constant2 : Constant  Value=TIMEOUT
  Constant3 : Constant  Value=T_STEP
  Gain : Gain  Gain=0
  Min1 : MinMax  Function=max  Inputs=2
  Min2 : MinMax  Inputs=2
  Relational Operator : RelationalOperator  Operator=>  OutDataTypeStr=boolean  RndMeth=Simplest
  Sum1 : Sum  Inputs=|++
  Sum2 : Sum  Inputs=|++
  Switch : Switch  Criteria=u2 > Threshold
  Unit Delay : UnitDelay  SampleTime=T_STEP
  out : Outport  VectorParamsAs1DForOutWhenUnconnected=on
  wires:
  Sum2/1 -> Relational Operator/1, Min2/1
  Sum1/1 -> Min2/2, Relational Operator/2
  Constant/1 -> Sum2/1
  Min2/1 -> Switch/1
  Constant1/1 -> Switch/3
  Unit Delay/1 -> Sum2/2
  in/1 -> Switch/2
  Switch/1 -> Unit Delay/1
  Relational Operator/1 -> out/1
  Min1/1 -> Sum1/1
  Constant2/1 -> Min1/1
  Constant3/1 -> Min1/2, Gain/1
  Gain/1 -> Sum1/2

== system My_gfm_battery_sil_1_BS_2/My Inverter Controller /My_acChecks_A_V2/UV3 Timer ==
  note: Min one sample delay on Rise
  note: Max one sample delay on Fall
  in : Inport
  Constant : Constant  Value=T_STEP
  Constant1 : Constant  Value=0
  Constant2 : Constant  Value=TIMEOUT
  Constant3 : Constant  Value=T_STEP
  Gain : Gain  Gain=0
  Min1 : MinMax  Function=max  Inputs=2
  Min2 : MinMax  Inputs=2
  Relational Operator : RelationalOperator  Operator=>  OutDataTypeStr=boolean  RndMeth=Simplest
  Sum1 : Sum  Inputs=|++
  Sum2 : Sum  Inputs=|++
  Switch : Switch  Criteria=u2 > Threshold
  Unit Delay : UnitDelay  SampleTime=T_STEP
  out : Outport  VectorParamsAs1DForOutWhenUnconnected=on
  wires:
  Sum2/1 -> Relational Operator/1, Min2/1
  Sum1/1 -> Min2/2, Relational Operator/2
  Constant/1 -> Sum2/1
  Min2/1 -> Switch/1
  Constant1/1 -> Switch/3
  Unit Delay/1 -> Sum2/2
  in/1 -> Switch/2
  Switch/1 -> Unit Delay/1
  Relational Operator/1 -> out/1
  Min1/1 -> Sum1/1
  Constant2/1 -> Min1/1
  Constant3/1 -> Min1/2, Gain/1
  Gain/1 -> Sum1/2

== system My_gfm_battery_sil_1_BS_2/My Inverter Controller /My_acChecks_A_V3/Assert Timer ==
  note: Min one sample delay on Rise
  note: Max one sample delay on Fall
  in : Inport
  Constant : Constant  Value=T_STEP
  Constant1 : Constant  Value=0
  Constant2 : Constant  Value=TIMEOUT
  Constant3 : Constant  Value=T_STEP
  Gain : Gain  Gain=0
  Min1 : MinMax  Function=max  Inputs=2
  Min2 : MinMax  Inputs=2
  Relational Operator : RelationalOperator  Operator=>  OutDataTypeStr=boolean  RndMeth=Simplest
  Sum1 : Sum  Inputs=|++
  Sum2 : Sum  Inputs=|++
  Switch : Switch  Criteria=u2 > Threshold
  Unit Delay : UnitDelay  SampleTime=T_STEP
  out : Outport  VectorParamsAs1DForOutWhenUnconnected=on
  wires:
  Sum2/1 -> Relational Operator/1, Min2/1
  Sum1/1 -> Min2/2, Relational Operator/2
  Constant/1 -> Sum2/1
  Min2/1 -> Switch/1
  Constant1/1 -> Switch/3
  Unit Delay/1 -> Sum2/2
  in/1 -> Switch/2
  Switch/1 -> Unit Delay/1
  Relational Operator/1 -> out/1
  Min1/1 -> Sum1/1
  Constant2/1 -> Min1/1
  Constant3/1 -> Min1/2, Gain/1
  Gain/1 -> Sum1/2

== system My_gfm_battery_sil_1_BS_2/My Inverter Controller /My_acChecks_A_V3/Assert Timer1 ==
  note: Min one sample delay on Rise
  note: Max one sample delay on Fall
  in : Inport
  Constant : Constant  Value=T_STEP
  Constant1 : Constant  Value=0
  Constant2 : Constant  Value=TIMEOUT
  Constant3 : Constant  Value=T_STEP
  Gain : Gain  Gain=0
  Min1 : MinMax  Function=max  Inputs=2
  Min2 : MinMax  Inputs=2
  Relational Operator : RelationalOperator  Operator=>  OutDataTypeStr=boolean  RndMeth=Simplest
  Sum1 : Sum  Inputs=|++
  Sum2 : Sum  Inputs=|++
  Switch : Switch  Criteria=u2 > Threshold
  Unit Delay : UnitDelay  SampleTime=T_STEP
  out : Outport  VectorParamsAs1DForOutWhenUnconnected=on
  wires:
  Sum2/1 -> Relational Operator/1, Min2/1
  Sum1/1 -> Min2/2, Relational Operator/2
  Constant/1 -> Sum2/1
  Min2/1 -> Switch/1
  Constant1/1 -> Switch/3
  Unit Delay/1 -> Sum2/2
  in/1 -> Switch/2
  Switch/1 -> Unit Delay/1
  Relational Operator/1 -> out/1
  Min1/1 -> Sum1/1
  Constant2/1 -> Min1/1
  Constant3/1 -> Min1/2, Gain/1
  Gain/1 -> Sum1/2

== system My_gfm_battery_sil_1_BS_2/My Inverter Controller /My_acChecks_A_V3/BS Assert Timer ==
  note: Min one sample delay on Rise
  note: Max one sample delay on Fall
  in : Inport
  Constant : Constant  Value=T_STEP
  Constant1 : Constant  Value=0
  Constant2 : Constant  Value=TIMEOUT
  Constant3 : Constant  Value=T_STEP
  Gain : Gain  Gain=0
  Min1 : MinMax  Function=max  Inputs=2
  Min2 : MinMax  Inputs=2
  Relational Operator : RelationalOperator  Operator=>  OutDataTypeStr=boolean  RndMeth=Simplest
  Sum1 : Sum  Inputs=|++
  Sum2 : Sum  Inputs=|++
  Switch : Switch  Criteria=u2 > Threshold
  Unit Delay : UnitDelay  SampleTime=T_STEP
  out : Outport  VectorParamsAs1DForOutWhenUnconnected=on
  wires:
  Sum2/1 -> Relational Operator/1, Min2/1
  Sum1/1 -> Min2/2, Relational Operator/2
  Constant/1 -> Sum2/1
  Min2/1 -> Switch/1
  Constant1/1 -> Switch/3
  Unit Delay/1 -> Sum2/2
  in/1 -> Switch/2
  Switch/1 -> Unit Delay/1
  Relational Operator/1 -> out/1
  Min1/1 -> Sum1/1
  Constant2/1 -> Min1/1
  Constant3/1 -> Min1/2, Gain/1
  Gain/1 -> Sum1/2

== system My_gfm_battery_sil_1_BS_2/My Inverter Controller /My_acChecks_A_V3/Clear Timer1 ==
  note: Max one sample delay on Rise
  note: Min one sample delay on Fall
  in : Inport
  Constant : Constant  Value=T_STEP
  Constant1 : Constant  Value=0
  Constant2 : Constant  Value=TIMEOUT
  Constant3 : Constant  Value=T_STEP
  Min1 : MinMax  Function=max  Inputs=2
  Min2 : MinMax  Function=max  Inputs=2
  Relational Operator : RelationalOperator  Operator=>  OutDataTypeStr=boolean  RndMeth=Simplest
  Sum1 : Sum  Inputs=|++
  Sum2 : Sum  Inputs=|-+
  Switch : Switch  Criteria=u2 > Threshold
  Unit Delay : UnitDelay  InitialCondition=TIMER_INIT  SampleTime=T_STEP
  out : Outport  VectorParamsAs1DForOutWhenUnconnected=on
  wires:
  Sum1/1 -> Switch/1
  Sum2/1 -> Relational Operator/1, Min2/1
  Constant/1 -> Sum2/1
  Min2/1 -> Switch/3
  Constant1/1 -> Min2/2, Relational Operator/2
  Unit Delay/1 -> Sum2/2
  in/1 -> Switch/2
  Switch/1 -> Unit Delay/1
  Relational Operator/1 -> out/1
  Constant2/1 -> Min1/1
  Constant3/1 -> Min1/2, Sum1/2
  Min1/1 -> Sum1/1

== system My_gfm_battery_sil_1_BS_2/My Inverter Controller /My_acChecks_A_V3/Clear Timer10 ==
  note: Max one sample delay on Rise
  note: Min one sample delay on Fall
  in : Inport
  Constant : Constant  Value=T_STEP
  Constant1 : Constant  Value=0
  Constant2 : Constant  Value=TIMEOUT
  Constant3 : Constant  Value=T_STEP
  Min1 : MinMax  Function=max  Inputs=2
  Min2 : MinMax  Function=max  Inputs=2
  Relational Operator : RelationalOperator  Operator=>  OutDataTypeStr=boolean  RndMeth=Simplest
  Sum1 : Sum  Inputs=|++
  Sum2 : Sum  Inputs=|-+
  Switch : Switch  Criteria=u2 > Threshold
  Unit Delay : UnitDelay  InitialCondition=TIMER_INIT  SampleTime=T_STEP
  out : Outport  VectorParamsAs1DForOutWhenUnconnected=on
  wires:
  Sum1/1 -> Switch/1
  Sum2/1 -> Relational Operator/1, Min2/1
  Constant/1 -> Sum2/1
  Min2/1 -> Switch/3
  Constant1/1 -> Min2/2, Relational Operator/2
  Unit Delay/1 -> Sum2/2
  in/1 -> Switch/2
  Switch/1 -> Unit Delay/1
  Relational Operator/1 -> out/1
  Constant2/1 -> Min1/1
  Constant3/1 -> Min1/2, Sum1/2
  Min1/1 -> Sum1/1

== system My_gfm_battery_sil_1_BS_2/My Inverter Controller /My_acChecks_A_V3/Clear Timer11 ==
  note: Max one sample delay on Rise
  note: Min one sample delay on Fall
  in : Inport
  Constant : Constant  Value=T_STEP
  Constant1 : Constant  Value=0
  Constant2 : Constant  Value=TIMEOUT
  Constant3 : Constant  Value=T_STEP
  Min1 : MinMax  Function=max  Inputs=2
  Min2 : MinMax  Function=max  Inputs=2
  Relational Operator : RelationalOperator  Operator=>  OutDataTypeStr=boolean  RndMeth=Simplest
  Sum1 : Sum  Inputs=|++
  Sum2 : Sum  Inputs=|-+
  Switch : Switch  Criteria=u2 > Threshold
  Unit Delay : UnitDelay  InitialCondition=TIMER_INIT  SampleTime=T_STEP
  out : Outport  VectorParamsAs1DForOutWhenUnconnected=on
  wires:
  Sum1/1 -> Switch/1
  Sum2/1 -> Relational Operator/1, Min2/1
  Constant/1 -> Sum2/1
  Min2/1 -> Switch/3
  Constant1/1 -> Min2/2, Relational Operator/2
  Unit Delay/1 -> Sum2/2
  in/1 -> Switch/2
  Switch/1 -> Unit Delay/1
  Relational Operator/1 -> out/1
  Constant2/1 -> Min1/1
  Constant3/1 -> Min1/2, Sum1/2
  Min1/1 -> Sum1/1

== system My_gfm_battery_sil_1_BS_2/My Inverter Controller /My_acChecks_A_V3/Clear Timer12 ==
  note: Max one sample delay on Rise
  note: Min one sample delay on Fall
  in : Inport
  Constant : Constant  Value=T_STEP
  Constant1 : Constant  Value=0
  Constant2 : Constant  Value=TIMEOUT
  Constant3 : Constant  Value=T_STEP
  Min1 : MinMax  Function=max  Inputs=2
  Min2 : MinMax  Function=max  Inputs=2
  Relational Operator : RelationalOperator  Operator=>  OutDataTypeStr=boolean  RndMeth=Simplest
  Sum1 : Sum  Inputs=|++
  Sum2 : Sum  Inputs=|-+
  Switch : Switch  Criteria=u2 > Threshold
  Unit Delay : UnitDelay  InitialCondition=TIMER_INIT  SampleTime=T_STEP
  out : Outport  VectorParamsAs1DForOutWhenUnconnected=on
  wires:
  Sum1/1 -> Switch/1
  Sum2/1 -> Relational Operator/1, Min2/1
  Constant/1 -> Sum2/1
  Min2/1 -> Switch/3
  Constant1/1 -> Min2/2, Relational Operator/2
  Unit Delay/1 -> Sum2/2
  in/1 -> Switch/2
  Switch/1 -> Unit Delay/1
  Relational Operator/1 -> out/1
  Constant2/1 -> Min1/1
  Constant3/1 -> Min1/2, Sum1/2
  Min1/1 -> Sum1/1

== system My_gfm_battery_sil_1_BS_2/My Inverter Controller /My_acChecks_A_V3/Clear Timer13 ==
  note: Max one sample delay on Rise
  note: Min one sample delay on Fall
  in : Inport
  Constant : Constant  Value=T_STEP
  Constant1 : Constant  Value=0
  Constant2 : Constant  Value=TIMEOUT
  Constant3 : Constant  Value=T_STEP
  Min1 : MinMax  Function=max  Inputs=2
  Min2 : MinMax  Function=max  Inputs=2
  Relational Operator : RelationalOperator  Operator=>  OutDataTypeStr=boolean  RndMeth=Simplest
  Sum1 : Sum  Inputs=|++
  Sum2 : Sum  Inputs=|-+
  Switch : Switch  Criteria=u2 > Threshold
  Unit Delay : UnitDelay  InitialCondition=TIMER_INIT  SampleTime=T_STEP
  out : Outport  VectorParamsAs1DForOutWhenUnconnected=on
  wires:
  Sum1/1 -> Switch/1
  Sum2/1 -> Relational Operator/1, Min2/1
  Constant/1 -> Sum2/1
  Min2/1 -> Switch/3
  Constant1/1 -> Min2/2, Relational Operator/2
  Unit Delay/1 -> Sum2/2
  in/1 -> Switch/2
  Switch/1 -> Unit Delay/1
  Relational Operator/1 -> out/1
  Constant2/1 -> Min1/1
  Constant3/1 -> Min1/2, Sum1/2
  Min1/1 -> Sum1/1

== system My_gfm_battery_sil_1_BS_2/My Inverter Controller /My_acChecks_A_V3/Clear Timer14 ==
  note: Max one sample delay on Rise
  note: Min one sample delay on Fall
  in : Inport
  Constant : Constant  Value=T_STEP
  Constant1 : Constant  Value=0
  Constant2 : Constant  Value=TIMEOUT
  Constant3 : Constant  Value=T_STEP
  Min1 : MinMax  Function=max  Inputs=2
  Min2 : MinMax  Function=max  Inputs=2
  Relational Operator : RelationalOperator  Operator=>  OutDataTypeStr=boolean  RndMeth=Simplest
  Sum1 : Sum  Inputs=|++
  Sum2 : Sum  Inputs=|-+
  Switch : Switch  Criteria=u2 > Threshold
  Unit Delay : UnitDelay  InitialCondition=TIMER_INIT  SampleTime=T_STEP
  out : Outport  VectorParamsAs1DForOutWhenUnconnected=on
  wires:
  Sum1/1 -> Switch/1
  Sum2/1 -> Relational Operator/1, Min2/1
  Constant/1 -> Sum2/1
  Min2/1 -> Switch/3
  Constant1/1 -> Min2/2, Relational Operator/2
  Unit Delay/1 -> Sum2/2
  in/1 -> Switch/2
  Switch/1 -> Unit Delay/1
  Relational Operator/1 -> out/1
  Constant2/1 -> Min1/1
  Constant3/1 -> Min1/2, Sum1/2
  Min1/1 -> Sum1/1

== system My_gfm_battery_sil_1_BS_2/My Inverter Controller /My_acChecks_A_V3/Clear Timer15 ==
  note: Max one sample delay on Rise
  note: Min one sample delay on Fall
  in : Inport
  Constant : Constant  Value=T_STEP
  Constant1 : Constant  Value=0
  Constant2 : Constant  Value=TIMEOUT
  Constant3 : Constant  Value=T_STEP
  Min1 : MinMax  Function=max  Inputs=2
  Min2 : MinMax  Function=max  Inputs=2
  Relational Operator : RelationalOperator  Operator=>  OutDataTypeStr=boolean  RndMeth=Simplest
  Sum1 : Sum  Inputs=|++
  Sum2 : Sum  Inputs=|-+
  Switch : Switch  Criteria=u2 > Threshold
  Unit Delay : UnitDelay  InitialCondition=TIMER_INIT  SampleTime=T_STEP
  out : Outport  VectorParamsAs1DForOutWhenUnconnected=on
  wires:
  Sum1/1 -> Switch/1
  Sum2/1 -> Relational Operator/1, Min2/1
  Constant/1 -> Sum2/1
  Min2/1 -> Switch/3
  Constant1/1 -> Min2/2, Relational Operator/2
  Unit Delay/1 -> Sum2/2
  in/1 -> Switch/2
  Switch/1 -> Unit Delay/1
  Relational Operator/1 -> out/1
  Constant2/1 -> Min1/1
  Constant3/1 -> Min1/2, Sum1/2
  Min1/1 -> Sum1/1
